simulink model "flex_afe_acquisition"  (R2024b)
settings: Solver=VariableStepAuto  StartTime=0.0  StopTime=5  RelTol=1e-3  AbsTol=1e-3
undefined symbols (not defined in the file): R_adc_in, R_div, R_filt, Ts
libraries: fl_lib x18, nesl_utility x4, simulink x1
settings Model: Creator=DELL  LastModifiedBy=DELL
settings SolverCC: AutoScaleAbsTol=off  AlgebraicLoopSolver=TrustRegion  MaxZcPerStep=1
settings DebuggingCC: UnconnectedInputMsg=warning  UnconnectedOutputMsg=warning  UnconnectedLineMsg=warning  SymbolicDimsDataTypeCodeGenerationDiagnostic=none
settings ModelReferenceCC: EnableRefExpFcnMdlSchedulingChecks=on
settings SFSimCC: CustomCodeUndefinedFunction=UseInterfaceOnly
settings RTWCC: GPUComputeCapability=3.5  DLArmComputeVersion=19.05
settings SimscapeCC: SimscapeLogType=all  SimscapeLogSimulationStatistics=on  SimscapeLogDataHistory=10000

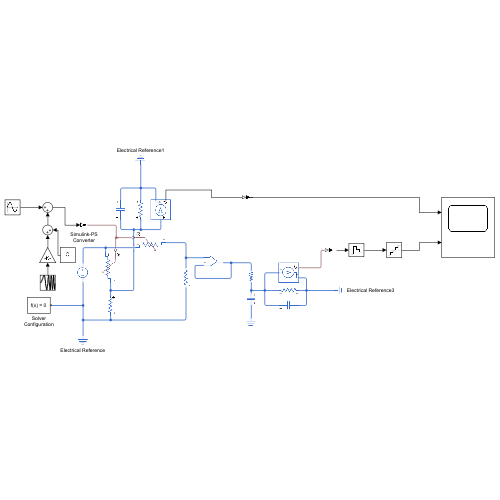
[thumbnail: Simulink's stored preview of the top-level diagram]
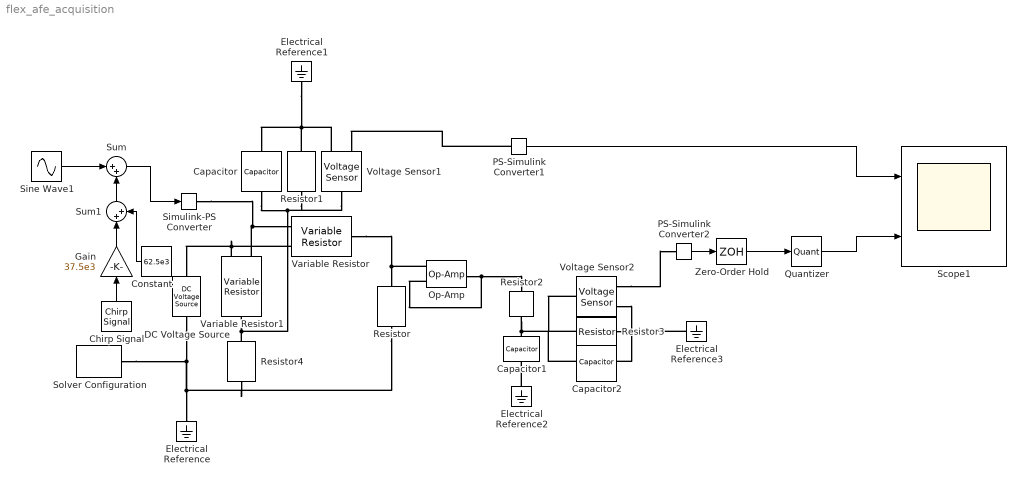
== system flex_afe_acquisition ==
  Capacitor : fl_lib/Electrical/Electrical Elements/Capacitor  c=C_sh F  r=1e-6 Ohm  g=0 1/Ohm  i_specify=off  i_priority=None  i=0 A  i_nominal_specify=off  i_nominal_value=1  i_nominal_unit=A  v_specify=off  v_priority=None  v=0 V  v_nominal_specify=off  v_nominal_value=1  v_nominal_unit=V  vc_specify=off  vc_priority=High  vc=0 V  vc_nominal_specify=off  vc_nominal_value=1  vc_nominal_unit=V
  Capacitor1 : fl_lib/Electrical/Electrical Elements/Capacitor  c=C_filt F  r=1e-6 Ohm  g=0 1/Ohm  i_specify=off  i_priority=None  i=0 A  i_nominal_specify=off  i_nominal_value=1  i_nominal_unit=A  v_specify=off  v_priority=None  v=0 V  v_nominal_specify=off  v_nominal_value=1  v_nominal_unit=V  vc_specify=off  vc_priority=High  vc=0 V  vc_nominal_specify=off  vc_nominal_value=1  vc_nominal_unit=V
  Capacitor2 : fl_lib/Electrical/Electrical Elements/Capacitor  c=C_sh F  r=1e-6 Ohm  g=0 1/Ohm  i_specify=off  i_priority=None  i=0 A  i_nominal_specify=off  i_nominal_value=1  i_nominal_unit=A  v_specify=off  v_priority=None  v=0 V  v_nominal_specify=off  v_nominal_value=1  v_nominal_unit=V  vc_specify=off  vc_priority=High  vc=0 V  vc_nominal_specify=off  vc_nominal_value=1  vc_nominal_unit=V
  Chirp Signal : simulink/Sources/Chirp Signal  f1=0.5  T=5  f2=15
  Constant : Constant  Value=62.5e3
  DC Voltage Source : fl_lib/Electrical/Electrical Sources/DC Voltage Source  v0=V_dd V
  Electrical Reference{,1..3} (4 alike) : fl_lib/Electrical/Electrical Elements/Electrical Reference
  Gain : Gain  Gain=37.5e3
  Op-Amp : fl_lib/Electrical/Electrical Elements/Op-Amp  outI_specify=off  outI_priority=None  outI=0 A  outI_nominal_specify=off  outI_nominal_value=1  outI_nominal_unit=A
  PS-Simulink Converter1 : nesl_utility/PS-Simulink Converter  PhysicalDomain=network_engine_domain  SubClassName=ps_output  LeftPortType=input  RightPortType=output  PseudoPeriodic=off  Frequencies=[]  VectorFormat=inherit  Unit=inherit  AffineConversion=off
  PS-Simulink Converter2 : nesl_utility/PS-Simulink Converter  PhysicalDomain=network_engine_domain  SubClassName=ps_output  LeftPortType=input  RightPortType=output  PseudoPeriodic=off  Frequencies=[]  VectorFormat=inherit  Unit=inherit  AffineConversion=off
  Quantizer : Quantizer  QuantizationInterval=adc_lsb
  Resistor : fl_lib/Electrical/Electrical Elements/Resistor  R=R_div Ohm  i_specify=off  i_priority=None  i=0 A  i_nominal_specify=off  i_nominal_value=1  i_nominal_unit=A  v_specify=off  v_priority=None  v=0 V  v_nominal_specify=off  v_nominal_value=1  v_nominal_unit=V
  Resistor1 : fl_lib/Electrical/Electrical Elements/Resistor  R=R_adc_in Ohm  i_specify=off  i_priority=None  i=0 A  i_nominal_specify=off  i_nominal_value=1  i_nominal_unit=A  v_specify=off  v_priority=None  v=0 V  v_nominal_specify=off  v_nominal_value=1  v_nominal_unit=V
  Resistor2 : fl_lib/Electrical/Electrical Elements/Resistor  R=R_filt Ohm  i_specify=off  i_priority=None  i=0 A  i_nominal_specify=off  i_nominal_value=1  i_nominal_unit=A  v_specify=off  v_priority=None  v=0 V  v_nominal_specify=off  v_nominal_value=1  v_nominal_unit=V
  Resistor3 : fl_lib/Electrical/Electrical Elements/Resistor  R=R_adc_in Ohm  i_specify=off  i_priority=None  i=0 A  i_nominal_specify=off  i_nominal_value=1  i_nominal_unit=A  v_specify=off  v_priority=None  v=0 V  v_nominal_specify=off  v_nominal_value=1  v_nominal_unit=V
  Resistor4 : fl_lib/Electrical/Electrical Elements/Resistor  R=R_div Ohm  i_specify=off  i_priority=None  i=0 A  i_nominal_specify=off  i_nominal_value=1  i_nominal_unit=A  v_specify=off  v_priority=None  v=0 V  v_nominal_specify=off  v_nominal_value=1  v_nominal_unit=V
  Scope1 : Scope  NumInputPorts=2
  Simulink-PS Converter : nesl_utility/Simulink-PS Converter  PhysicalDomain=network_engine_domain  SubClassName=ps_input  LeftPortType=input  RightPortType=output  PseudoPeriodic=off  Frequencies=[]  NoiseDistribution=none  NoiseParameters=[]  Unit=1  AffineConversion=off  FilteringAndDerivatives=filter  SimscapeFilterOrder=1  InputFilterTimeConstant=0.001  UdotUserProvided=0
  Sine Wave1 : Sin  Amplitude=2e3  Frequency=2*pi*50  SampleTime=0
  Solver Configuration : nesl_utility/Solver Configuration  PhysicalDomain=network_engine_domain  SubClassName=solver  LeftPortType=input  RightPortType=generic  Tones=[]  Harmonics=[]  SimulateNoise=off  Profile=off  UseLocalSampling=off  EnableSwitchedLinearOptims=on  FrequencyDomain=off  UseCCode=off  RelTol=0.001  AbsTol=1e-06  MinStep=1e-09  ToWorkspace=off  RevertToSquareIcSolve=off  NumHomotopyIterations=100  PhasorMode=off  PhasorModeNumHarmonics=1  ConsistencySolver=NEWTON_XTOL_AFTER_FTOL  IndexReductionMethod=DerivativeReplacement  DoDC=off  ResidualTolerance=1e-09  ConsistencyTolSource=GLOBAL  ConsistencyAbsTol=0.001  ConsistencyRelTol=0.001  ConsistencyTolFactor=0.001  UseLocalSolver=off  LocalSolverChoice=NE_BACKWARD_EULER_ADVANCER  ResolveIndetEquations=on  FunctionEvalNumThread=1  LocalSolverSampleTime=0.001  DoFixedCost=off  MaxNonlinIter=3  MaxModeIter=2  ComputeImpulses=off  ImpulseIterations=2  LinearAlgebra=auto  LinearAlgebraNumThread=0  EquationFormulation=NE_TIME_EF  DelaysMemoryBudget=1024  AutomaticFiltering=on  FilteringTimeConstant=0.001  PartitionStorageMethod=AS_NEEDED  PartitionMemoryBudget=1024  PartitionMethod=ROBUST  MultibodyUseLocalSolver=off  MultibodyLocalSolverChoice=ODE1  MultibodyLocalSolverSampleTime=0.001
  Sum : Sum  Inputs=|++
  Sum1 : Sum  Inputs=|++
  Variable Resistor : fl_lib/Electrical/Electrical Elements/Variable Resistor  Rmin=R_flat Ohm  thermalEnable=false  thermal_mass=1 J/K  i_specify=off  i_priority=None  i=0 A  i_nominal_specify=off  i_nominal_value=1  i_nominal_unit=A  v_specify=off  v_priority=None  v=0 V  v_nominal_specify=off  v_nominal_value=1  v_nominal_unit=V  T_specify=off  T_priority=None  T=300 K  T_nominal_specify=off  T_nominal_value=1  T_nominal_unit=K
  Variable Resistor1 : fl_lib/Electrical/Electrical Elements/Variable Resistor  Rmin=R_flat Ohm  thermalEnable=false  thermal_mass=1 J/K  i_specify=off  i_priority=None  i=0 A  i_nominal_specify=off  i_nominal_value=1  i_nominal_unit=A  v_specify=off  v_priority=None  v=0 V  v_nominal_specify=off  v_nominal_value=1  v_nominal_unit=V  T_specify=off  T_priority=None  T=300 K  T_nominal_specify=off  T_nominal_value=1  T_nominal_unit=K
  Voltage Sensor1 : fl_lib/Electrical/Electrical Sensors/Voltage Sensor
  Voltage Sensor2 : fl_lib/Electrical/Electrical Sensors/Voltage Sensor
  Zero-Order Hold : ZeroOrderHold  SampleTime=Ts
  wires:
  PS-Simulink Converter2/1 -> Zero-Order Hold/1
  Sine Wave1/1 -> Sum/1
  Chirp Signal/1 -> Gain/1
  Sum/1 -> Simulink-PS Converter/1
  PS-Simulink Converter1/1 -> Scope1/1
  Zero-Order Hold/1 -> Quantizer/1
  Quantizer/1 -> Scope1/2
  Gain/1 -> Sum1/1
  Constant/1 -> Sum1/2
  Sum1/1 -> Sum/2
  connections:
  Solver Configuration/RConn1 -- Resistor4/RConn1 -- Resistor/RConn1 -- Electrical Reference/LConn1 -- DC Voltage Source/RConn1
  Variable Resistor/LConn2 -- Variable Resistor1/LConn2 -- DC Voltage Source/LConn1
  Simulink-PS Converter/RConn1 -- Variable Resistor1/LConn1 -- Variable Resistor/LConn1
  Variable Resistor/RConn1 -- Op-Amp/LConn1 -- Resistor/LConn1
  Resistor1/RConn1 -- Voltage Sensor1/RConn2 -- Capacitor/RConn1 -- Electrical Reference1/LConn1
  PS-Simulink Converter1/LConn1 -- Voltage Sensor1/RConn1
  Op-Amp/RConn1 -- Op-Amp/LConn2 -- Resistor2/LConn1
  Capacitor1/LConn1 -- Capacitor2/LConn1 -- Resistor3/LConn1 -- Voltage Sensor2/LConn1 -- Resistor2/RConn1
  Electrical Reference2/LConn1 -- Capacitor1/RConn1
  Electrical Reference3/LConn1 -- Capacitor2/RConn1 -- Resistor3/RConn1 -- Voltage Sensor2/RConn2
  Voltage Sensor2/RConn1 -- PS-Simulink Converter2/LConn1
  Resistor4/LConn1 -- Resistor1/LConn1 -- Voltage Sensor1/LConn1 -- Capacitor/LConn1 -- Variable Resistor1/RConn1
